simulink model "hdlcoder_nibbleswap_eml"  (R2026a)
settings: Solver=FixedStepDiscrete  StopTime=10  FixedStep=1
settings Model: Creator=The MathWorks, Inc.  LastModifiedBy=The MathWorks, Inc.
settings OptimizationCC: ConditionallyExecuteInputs=off  InitFltsAndDblsToZero=on
settings DebuggingCC: AlgebraicLoopMsg=error  UnderspecifiedInitializationDetection=Classic  MultiTaskDSMMsg=warning  MultiTaskCondExecSysMsg=none  SingleTaskRateTransMsg=error
settings HardwareCC: ProdHWDeviceType=ASIC/FPGA  ProdEqTarget=off
settings GRTTargetCC: TargetFcnLib=ansi_tfl_tmw_new.mat  CombineOutputUpdateFcns=off  GRTInterface=on

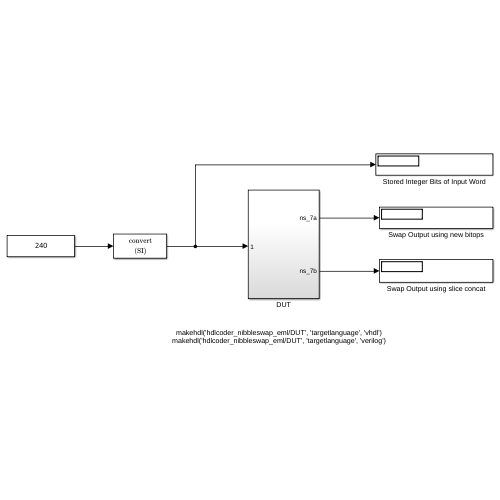
[thumbnail: Simulink's stored preview of the top-level diagram]
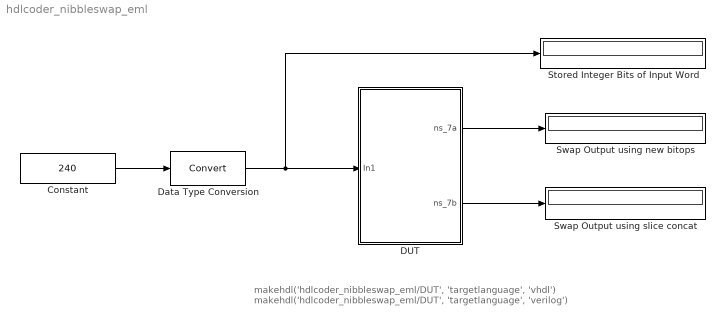
== system hdlcoder_nibbleswap_eml ==
  note: makehdl('hdlcoder_nibbleswap_eml/DUT', 'targetlanguage', 'vhdl')
      | makehdl('hdlcoder_nibbleswap_eml/DUT', 'targetlanguage', 'verilog')
  Constant : Constant  Value=240  SampleTime=1
  DUT : Subsystem
  Data Type Conversion : DataTypeConversion  ConvertRealWorld=Stored Integer (SI)  SaturateOnIntegerOverflow=off  RndMeth=Floor
  Stored Integer Bits of Input Word : Display
      settings: Format=binary (Stored Integer)
  Swap Output using new bitops : Display
      settings: Format=binary (Stored Integer)
  Swap Output using slice concat : Display
      settings: Format=binary (Stored Integer)
  wires:
  Constant/1 -> Data Type Conversion/1
  Data Type Conversion/1 -> DUT/1(In1), Stored Integer Bits of Input Word/1
  DUT/1(ns_7a) -> Swap Output using new bitops/1
  DUT/2(ns_7b) -> Swap Output using slice concat/1

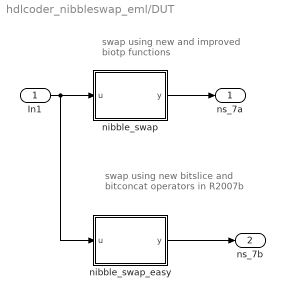
== system hdlcoder_nibbleswap_eml/DUT ==
  note: swap using new and improved
      | biotp functions
  note: swap using new
      | bitslice and bitconcat operators
      | in R2007b
  In1 : Inport
  nibble_swap : MATLAB Function  TreatAsAtomicUnit=on
  nibble_swap_easy : MATLAB Function  TreatAsAtomicUnit=on
  ns_7a : Outport
  ns_7b : Outport  Port=2
  wires:
  In1/1 -> nibble_swap_easy/1(u), nibble_swap/1(u)
  nibble_swap/1(y) -> ns_7a/1
  nibble_swap_easy/1(y) -> ns_7b/1

== matlab function hdlcoder_nibbleswap_eml/DUT/nibble_swap_easy ==
  settings: fimath=|
      | fimath(...
      | 'RoundMode', 'floor',...
      | 'OverflowMode', 'wrap',...
      | 'ProductMode', 'FullPrecision', 'ProductWordLength', 32,...
      | 'SumMode', 'FullPrecision', 'SumWordLength', 32,...
      | 'CastBeforeSum', true)
  data: u input fixdt(0,8,0); y output
function y = fcn(u)
% NIBBLE SWAP
y = bitconcat(bitsliceget(u, uint8(4), uint8(1)), bitsliceget(u, uint8(8),uint8(5)));

== matlab function hdlcoder_nibbleswap_eml/DUT/nibble_swap ==
  settings: fimath=|
      | fimath(...
      | 'RoundMode', 'floor',...
      | 'OverflowMode', 'wrap',...
      | 'ProductMode', 'FullPrecision', 'ProductWordLength', 32,...
      | 'SumMode', 'FullPrecision', 'SumWordLength', 32,...
      | 'CastBeforeSum', true)
  data: u input fixdt(0,8,0); y output
function y = fcn(u)
% NIBBLE SWAP

% assumes u is of type ufix8
% lmask = 0x0F
lmask = fi(15, 0, 8, 0, 'fimath', fimath(u));

% lmask = 0xF0
umask = bitsll(lmask, 4);

% mask upper nibble
l_nibble = bitand(u, lmask);

% mask lower nibble
u_nibble = bitand(u, umask);

% shift lower nibble left
ls = bitsll(l_nibble, 4);

% shift upper nibble right
ur = bitsrl(u_nibble, 4);

% final output
y = bitor(ls, ur);
